simulink library "xps_library"  (Simulink 8.0)
settings: Solver=ode45  SolverMode=SingleTasking  StartTime=0.0  StopTime=10.0  RelTol=1e-3
undefined symbols (not defined in the file): sys_clk, xps_library_software_register_user_data_in
libraries: xbsIndex_r4 x867, simulink x109, dspsigops x81, casper_library_flow_control x68, xps_library x18, casper_library_misc x11
(part 10 of 10)

== system xps_library/DACs/dac_mkid/Subsystem/parallel_to_serial_converter ==
  pin : Inport
  ld : Inport  Port=2
  shift : Inport  Port=3
  Logical : xbsIndex_r4/Logical  logical_function=OR  inputs=2  en=off  latency=0  precision=Full  arith_type=Unsigned  n_bits=16  bin_pt=0  align_bp=on  dbl_ovrd=off  block_type=logical
  filler : xbsIndex_r4/Constant  const=0  gui_display_data_type=Fixed-point  arith_type=Unsigned  n_bits=sout_width  bin_pt=0  preci_type=Single  exp_width=8  frac_width=24  explicit_period=on  period=1  equ=P=C  opselect=C  inp2=PCIN>>17  opr=+  inp1=P  carry=CIN  dbl_ovrd=off  block_type=constant
  shifter_unit1 : casper_library_flow_control/shifter_unit  data_width=1  pin_offset=0
  shifter_unit10 : casper_library_flow_control/shifter_unit  data_width=1  pin_offset=9
  shifter_unit11 : casper_library_flow_control/shifter_unit  data_width=1  pin_offset=10
  shifter_unit12 : casper_library_flow_control/shifter_unit  data_width=1  pin_offset=11
  shifter_unit13 : casper_library_flow_control/shifter_unit  data_width=1  pin_offset=12
  shifter_unit14 : casper_library_flow_control/shifter_unit  data_width=1  pin_offset=13
  shifter_unit15 : casper_library_flow_control/shifter_unit  data_width=1  pin_offset=14
  shifter_unit16 : casper_library_flow_control/shifter_unit  data_width=1  pin_offset=15
  shifter_unit17 : casper_library_flow_control/shifter_unit  data_width=1  pin_offset=16
  shifter_unit2 : casper_library_flow_control/shifter_unit  data_width=1  pin_offset=1
  shifter_unit3 : casper_library_flow_control/shifter_unit  data_width=1  pin_offset=2
  shifter_unit4 : casper_library_flow_control/shifter_unit  data_width=1  pin_offset=3
  shifter_unit5 : casper_library_flow_control/shifter_unit  data_width=1  pin_offset=4
  shifter_unit6 : casper_library_flow_control/shifter_unit  data_width=1  pin_offset=5
  shifter_unit7 : casper_library_flow_control/shifter_unit  data_width=1  pin_offset=6
  shifter_unit8 : casper_library_flow_control/shifter_unit  data_width=1  pin_offset=7
  shifter_unit9 : casper_library_flow_control/shifter_unit  data_width=1  pin_offset=8
  sout : Outport
  wires:
  ld/1 -> Logical/1, shifter_unit1/1, shifter_unit2/1, shifter_unit3/1, shifter_unit4/1, shifter_unit5/1, shifter_unit6/1, shifter_unit7/1, shifter_unit8/1, shifter_unit9/1, shifter_unit10/1, shifter_unit11/1, shifter_unit12/1, shifter_unit13/1, shifter_unit14/1, shifter_unit15/1, shifter_unit16/1, shifter_unit17/1
  shift/1 -> Logical/2
  filler/1 -> shifter_unit1/2
  pin/1 -> shifter_unit1/3, shifter_unit2/3, shifter_unit3/3, shifter_unit4/3, shifter_unit5/3, shifter_unit6/3, shifter_unit7/3, shifter_unit8/3, shifter_unit9/3, shifter_unit10/3, shifter_unit11/3, shifter_unit12/3, shifter_unit13/3, shifter_unit14/3, shifter_unit15/3, shifter_unit16/3, shifter_unit17/3
  Logical/1 -> shifter_unit1/4, shifter_unit2/4, shifter_unit3/4, shifter_unit4/4, shifter_unit5/4, shifter_unit6/4, shifter_unit7/4, shifter_unit8/4, shifter_unit9/4, shifter_unit10/4, shifter_unit11/4, shifter_unit12/4, shifter_unit13/4, shifter_unit14/4, shifter_unit15/4, shifter_unit16/4, shifter_unit17/4
  shifter_unit1/1 -> shifter_unit2/2
  shifter_unit2/1 -> shifter_unit3/2
  shifter_unit3/1 -> shifter_unit4/2
  shifter_unit4/1 -> shifter_unit5/2
  shifter_unit5/1 -> shifter_unit6/2
  shifter_unit6/1 -> shifter_unit7/2
  shifter_unit7/1 -> shifter_unit8/2
  shifter_unit8/1 -> shifter_unit9/2
  shifter_unit9/1 -> shifter_unit10/2
  shifter_unit10/1 -> shifter_unit11/2
  shifter_unit11/1 -> shifter_unit12/2
  shifter_unit12/1 -> shifter_unit13/2
  shifter_unit13/1 -> shifter_unit14/2
  shifter_unit14/1 -> shifter_unit15/2
  shifter_unit15/1 -> shifter_unit16/2
  shifter_unit16/1 -> shifter_unit17/2
  shifter_unit17/1 -> sout/1

== system xps_library/DACs/dac_mkid/Subsystem/parallel_to_serial_converter1 ==
  pin : Inport
  ld : Inport  Port=2
  shift : Inport  Port=3
  Logical : xbsIndex_r4/Logical  logical_function=OR  inputs=2  en=off  latency=0  precision=Full  arith_type=Unsigned  n_bits=16  bin_pt=0  align_bp=on  dbl_ovrd=off  block_type=logical
  filler : xbsIndex_r4/Constant  const=0  gui_display_data_type=Fixed-point  arith_type=Unsigned  n_bits=sout_width  bin_pt=0  preci_type=Single  exp_width=8  frac_width=24  explicit_period=on  period=1  equ=P=C  opselect=C  inp2=PCIN>>17  opr=+  inp1=P  carry=CIN  dbl_ovrd=off  block_type=constant
  shifter_unit1 : casper_library_flow_control/shifter_unit  data_width=1  pin_offset=0
  shifter_unit10 : casper_library_flow_control/shifter_unit  data_width=1  pin_offset=9
  shifter_unit11 : casper_library_flow_control/shifter_unit  data_width=1  pin_offset=10
  shifter_unit12 : casper_library_flow_control/shifter_unit  data_width=1  pin_offset=11
  shifter_unit13 : casper_library_flow_control/shifter_unit  data_width=1  pin_offset=12
  shifter_unit14 : casper_library_flow_control/shifter_unit  data_width=1  pin_offset=13
  shifter_unit15 : casper_library_flow_control/shifter_unit  data_width=1  pin_offset=14
  shifter_unit16 : casper_library_flow_control/shifter_unit  data_width=1  pin_offset=15
  shifter_unit17 : casper_library_flow_control/shifter_unit  data_width=1  pin_offset=16
  shifter_unit2 : casper_library_flow_control/shifter_unit  data_width=1  pin_offset=1
  shifter_unit3 : casper_library_flow_control/shifter_unit  data_width=1  pin_offset=2
  shifter_unit4 : casper_library_flow_control/shifter_unit  data_width=1  pin_offset=3
  shifter_unit5 : casper_library_flow_control/shifter_unit  data_width=1  pin_offset=4
  shifter_unit6 : casper_library_flow_control/shifter_unit  data_width=1  pin_offset=5
  shifter_unit7 : casper_library_flow_control/shifter_unit  data_width=1  pin_offset=6
  shifter_unit8 : casper_library_flow_control/shifter_unit  data_width=1  pin_offset=7
  shifter_unit9 : casper_library_flow_control/shifter_unit  data_width=1  pin_offset=8
  sout : Outport
  wires:
  ld/1 -> Logical/1, shifter_unit1/1, shifter_unit2/1, shifter_unit3/1, shifter_unit4/1, shifter_unit5/1, shifter_unit6/1, shifter_unit7/1, shifter_unit8/1, shifter_unit9/1, shifter_unit10/1, shifter_unit11/1, shifter_unit12/1, shifter_unit13/1, shifter_unit14/1, shifter_unit15/1, shifter_unit16/1, shifter_unit17/1
  shift/1 -> Logical/2
  filler/1 -> shifter_unit1/2
  pin/1 -> shifter_unit1/3, shifter_unit2/3, shifter_unit3/3, shifter_unit4/3, shifter_unit5/3, shifter_unit6/3, shifter_unit7/3, shifter_unit8/3, shifter_unit9/3, shifter_unit10/3, shifter_unit11/3, shifter_unit12/3, shifter_unit13/3, shifter_unit14/3, shifter_unit15/3, shifter_unit16/3, shifter_unit17/3
  Logical/1 -> shifter_unit1/4, shifter_unit2/4, shifter_unit3/4, shifter_unit4/4, shifter_unit5/4, shifter_unit6/4, shifter_unit7/4, shifter_unit8/4, shifter_unit9/4, shifter_unit10/4, shifter_unit11/4, shifter_unit12/4, shifter_unit13/4, shifter_unit14/4, shifter_unit15/4, shifter_unit16/4, shifter_unit17/4
  shifter_unit1/1 -> shifter_unit2/2
  shifter_unit2/1 -> shifter_unit3/2
  shifter_unit3/1 -> shifter_unit4/2
  shifter_unit4/1 -> shifter_unit5/2
  shifter_unit5/1 -> shifter_unit6/2
  shifter_unit6/1 -> shifter_unit7/2
  shifter_unit7/1 -> shifter_unit8/2
  shifter_unit8/1 -> shifter_unit9/2
  shifter_unit9/1 -> shifter_unit10/2
  shifter_unit10/1 -> shifter_unit11/2
  shifter_unit11/1 -> shifter_unit12/2
  shifter_unit12/1 -> shifter_unit13/2
  shifter_unit13/1 -> shifter_unit14/2
  shifter_unit14/1 -> shifter_unit15/2
  shifter_unit15/1 -> shifter_unit16/2
  shifter_unit16/1 -> shifter_unit17/2
  shifter_unit17/1 -> sout/1

== system xps_library/DACs/dac_mkid/Subsystem/posedge1 ==
  In : Inport
  Delay : xbsIndex_r4/Delay  rst=off  infoeditControl=Selection of Reset will increase slice count due to use of real FFs and instead of SRLs  en=off  latency=1  dbl_ovrd=off  reg_retiming=off  block_type=delay
      settings: xl_area=[0, 0, 0, 0, 0, 0, 0]  block_version=9.1.01
  Inverter : xbsIndex_r4/Inverter  en=off  latency=0  dbl_ovrd=off  block_type=inv
      settings: xl_area=[0, 0, 0, 0, 0, 0, 0]  block_version=9.1.01
  Logical : xbsIndex_r4/Logical  logical_function=AND  inputs=2  en=off  latency=0  precision=Full  arith_type=Unsigned  n_bits=8  bin_pt=2  align_bp=on  dbl_ovrd=off  block_type=logical
      settings: xl_area=[0, 0, 0, 0, 0, 0, 0]  block_version=9.1.01
  Out : Outport
  wires:
  Delay/1 -> Inverter/1
  Inverter/1 -> Logical/1
  In/1 -> Delay/1, Logical/2
  Logical/1 -> Out/1

== system xps_library/DACs/dac_mkid/Subsystem/posedge2 ==
  In : Inport
  Delay : xbsIndex_r4/Delay  rst=off  infoeditControl=Selection of Reset will increase slice count due to use of real FFs and instead of SRLs  en=off  latency=1  dbl_ovrd=off  reg_retiming=off  block_type=delay
      settings: xl_area=[0, 0, 0, 0, 0, 0, 0]  block_version=9.1.01
  Inverter : xbsIndex_r4/Inverter  en=off  latency=0  dbl_ovrd=off  block_type=inv
      settings: xl_area=[0, 0, 0, 0, 0, 0, 0]  block_version=9.1.01
  Logical : xbsIndex_r4/Logical  logical_function=AND  inputs=2  en=off  latency=0  precision=Full  arith_type=Unsigned  n_bits=8  bin_pt=2  align_bp=on  dbl_ovrd=off  block_type=logical
      settings: xl_area=[0, 0, 0, 0, 0, 0, 0]  block_version=9.1.01
  Out : Outport
  wires:
  Delay/1 -> Inverter/1
  Inverter/1 -> Logical/1
  In/1 -> Delay/1, Logical/2
  Logical/1 -> Out/1

== system xps_library/DACs/dac_mkid/Subsystem/posedge3 ==
  In : Inport
  Delay : xbsIndex_r4/Delay  rst=off  infoeditControl=Selection of Reset will increase slice count due to use of real FFs and instead of SRLs  en=off  latency=1  dbl_ovrd=off  reg_retiming=off  block_type=delay
      settings: xl_area=[0, 0, 0, 0, 0, 0, 0]  block_version=9.1.01
  Inverter : xbsIndex_r4/Inverter  en=off  latency=0  dbl_ovrd=off  block_type=inv
      settings: xl_area=[0, 0, 0, 0, 0, 0, 0]  block_version=9.1.01
  Logical : xbsIndex_r4/Logical  logical_function=AND  inputs=2  en=off  latency=0  precision=Full  arith_type=Unsigned  n_bits=8  bin_pt=2  align_bp=on  dbl_ovrd=off  block_type=logical
      settings: xl_area=[0, 0, 0, 0, 0, 0, 0]  block_version=9.1.01
  Out : Outport
  wires:
  Delay/1 -> Inverter/1
  Inverter/1 -> Logical/1
  In/1 -> Delay/1, Logical/2
  Logical/1 -> Out/1

== system xps_library/DACs/dac_mkid_4x/Subsystem/parallel_to_serial_converter ==
  pin : Inport
  ld : Inport  Port=2
  shift : Inport  Port=3
  Logical : xbsIndex_r4/Logical  logical_function=OR  inputs=2  en=off  latency=0  precision=Full  arith_type=Unsigned  n_bits=16  bin_pt=0  align_bp=on  dbl_ovrd=off  block_type=logical
  filler : xbsIndex_r4/Constant  const=0  gui_display_data_type=Fixed-point  arith_type=Unsigned  n_bits=sout_width  bin_pt=0  preci_type=Single  exp_width=8  frac_width=24  explicit_period=on  period=1  equ=P=C  opselect=C  inp2=PCIN>>17  opr=+  inp1=P  carry=CIN  dbl_ovrd=off  block_type=constant
  shifter_unit1 : casper_library_flow_control/shifter_unit  data_width=1  pin_offset=0
  shifter_unit10 : casper_library_flow_control/shifter_unit  data_width=1  pin_offset=9
  shifter_unit11 : casper_library_flow_control/shifter_unit  data_width=1  pin_offset=10
  shifter_unit12 : casper_library_flow_control/shifter_unit  data_width=1  pin_offset=11
  shifter_unit13 : casper_library_flow_control/shifter_unit  data_width=1  pin_offset=12
  shifter_unit14 : casper_library_flow_control/shifter_unit  data_width=1  pin_offset=13
  shifter_unit15 : casper_library_flow_control/shifter_unit  data_width=1  pin_offset=14
  shifter_unit16 : casper_library_flow_control/shifter_unit  data_width=1  pin_offset=15
  shifter_unit17 : casper_library_flow_control/shifter_unit  data_width=1  pin_offset=16
  shifter_unit2 : casper_library_flow_control/shifter_unit  data_width=1  pin_offset=1
  shifter_unit3 : casper_library_flow_control/shifter_unit  data_width=1  pin_offset=2
  shifter_unit4 : casper_library_flow_control/shifter_unit  data_width=1  pin_offset=3
  shifter_unit5 : casper_library_flow_control/shifter_unit  data_width=1  pin_offset=4
  shifter_unit6 : casper_library_flow_control/shifter_unit  data_width=1  pin_offset=5
  shifter_unit7 : casper_library_flow_control/shifter_unit  data_width=1  pin_offset=6
  shifter_unit8 : casper_library_flow_control/shifter_unit  data_width=1  pin_offset=7
  shifter_unit9 : casper_library_flow_control/shifter_unit  data_width=1  pin_offset=8
  sout : Outport
  wires:
  shifter_unit17/1 -> sout/1
  shifter_unit16/1 -> shifter_unit17/2
  shifter_unit15/1 -> shifter_unit16/2
  shifter_unit14/1 -> shifter_unit15/2
  shifter_unit13/1 -> shifter_unit14/2
  shifter_unit12/1 -> shifter_unit13/2
  shifter_unit11/1 -> shifter_unit12/2
  shifter_unit10/1 -> shifter_unit11/2
  shifter_unit9/1 -> shifter_unit10/2
  shifter_unit8/1 -> shifter_unit9/2
  shifter_unit7/1 -> shifter_unit8/2
  shifter_unit6/1 -> shifter_unit7/2
  shifter_unit5/1 -> shifter_unit6/2
  shifter_unit4/1 -> shifter_unit5/2
  shifter_unit3/1 -> shifter_unit4/2
  shifter_unit2/1 -> shifter_unit3/2
  shifter_unit1/1 -> shifter_unit2/2
  Logical/1 -> shifter_unit17/4, shifter_unit16/4, shifter_unit15/4, shifter_unit14/4, shifter_unit13/4, shifter_unit12/4, shifter_unit11/4, shifter_unit10/4, shifter_unit9/4, shifter_unit8/4, shifter_unit7/4, shifter_unit6/4, shifter_unit5/4, shifter_unit4/4, shifter_unit3/4, shifter_unit2/4, shifter_unit1/4
  pin/1 -> shifter_unit17/3, shifter_unit16/3, shifter_unit15/3, shifter_unit14/3, shifter_unit13/3, shifter_unit12/3, shifter_unit11/3, shifter_unit10/3, shifter_unit9/3, shifter_unit8/3, shifter_unit7/3, shifter_unit6/3, shifter_unit5/3, shifter_unit4/3, shifter_unit3/3, shifter_unit2/3, shifter_unit1/3
  filler/1 -> shifter_unit1/2
  shift/1 -> Logical/2
  ld/1 -> shifter_unit17/1, shifter_unit16/1, shifter_unit15/1, shifter_unit14/1, shifter_unit13/1, shifter_unit12/1, shifter_unit11/1, shifter_unit10/1, shifter_unit9/1, shifter_unit8/1, shifter_unit7/1, shifter_unit6/1, shifter_unit5/1, shifter_unit4/1, shifter_unit3/1, shifter_unit2/1, shifter_unit1/1, Logical/1

== system xps_library/DACs/dac_mkid_4x/Subsystem/parallel_to_serial_converter1 ==
  pin : Inport
  ld : Inport  Port=2
  shift : Inport  Port=3
  Logical : xbsIndex_r4/Logical  logical_function=OR  inputs=2  en=off  latency=0  precision=Full  arith_type=Unsigned  n_bits=16  bin_pt=0  align_bp=on  dbl_ovrd=off  block_type=logical
  filler : xbsIndex_r4/Constant  const=0  gui_display_data_type=Fixed-point  arith_type=Unsigned  n_bits=sout_width  bin_pt=0  preci_type=Single  exp_width=8  frac_width=24  explicit_period=on  period=1  equ=P=C  opselect=C  inp2=PCIN>>17  opr=+  inp1=P  carry=CIN  dbl_ovrd=off  block_type=constant
  shifter_unit1 : casper_library_flow_control/shifter_unit  data_width=1  pin_offset=0
  shifter_unit10 : casper_library_flow_control/shifter_unit  data_width=1  pin_offset=9
  shifter_unit11 : casper_library_flow_control/shifter_unit  data_width=1  pin_offset=10
  shifter_unit12 : casper_library_flow_control/shifter_unit  data_width=1  pin_offset=11
  shifter_unit13 : casper_library_flow_control/shifter_unit  data_width=1  pin_offset=12
  shifter_unit14 : casper_library_flow_control/shifter_unit  data_width=1  pin_offset=13
  shifter_unit15 : casper_library_flow_control/shifter_unit  data_width=1  pin_offset=14
  shifter_unit16 : casper_library_flow_control/shifter_unit  data_width=1  pin_offset=15
  shifter_unit17 : casper_library_flow_control/shifter_unit  data_width=1  pin_offset=16
  shifter_unit2 : casper_library_flow_control/shifter_unit  data_width=1  pin_offset=1
  shifter_unit3 : casper_library_flow_control/shifter_unit  data_width=1  pin_offset=2
  shifter_unit4 : casper_library_flow_control/shifter_unit  data_width=1  pin_offset=3
  shifter_unit5 : casper_library_flow_control/shifter_unit  data_width=1  pin_offset=4
  shifter_unit6 : casper_library_flow_control/shifter_unit  data_width=1  pin_offset=5
  shifter_unit7 : casper_library_flow_control/shifter_unit  data_width=1  pin_offset=6
  shifter_unit8 : casper_library_flow_control/shifter_unit  data_width=1  pin_offset=7
  shifter_unit9 : casper_library_flow_control/shifter_unit  data_width=1  pin_offset=8
  sout : Outport
  wires:
  shifter_unit17/1 -> sout/1
  shifter_unit16/1 -> shifter_unit17/2
  shifter_unit15/1 -> shifter_unit16/2
  shifter_unit14/1 -> shifter_unit15/2
  shifter_unit13/1 -> shifter_unit14/2
  shifter_unit12/1 -> shifter_unit13/2
  shifter_unit11/1 -> shifter_unit12/2
  shifter_unit10/1 -> shifter_unit11/2
  shifter_unit9/1 -> shifter_unit10/2
  shifter_unit8/1 -> shifter_unit9/2
  shifter_unit7/1 -> shifter_unit8/2
  shifter_unit6/1 -> shifter_unit7/2
  shifter_unit5/1 -> shifter_unit6/2
  shifter_unit4/1 -> shifter_unit5/2
  shifter_unit3/1 -> shifter_unit4/2
  shifter_unit2/1 -> shifter_unit3/2
  shifter_unit1/1 -> shifter_unit2/2
  Logical/1 -> shifter_unit17/4, shifter_unit16/4, shifter_unit15/4, shifter_unit14/4, shifter_unit13/4, shifter_unit12/4, shifter_unit11/4, shifter_unit10/4, shifter_unit9/4, shifter_unit8/4, shifter_unit7/4, shifter_unit6/4, shifter_unit5/4, shifter_unit4/4, shifter_unit3/4, shifter_unit2/4, shifter_unit1/4
  pin/1 -> shifter_unit17/3, shifter_unit16/3, shifter_unit15/3, shifter_unit14/3, shifter_unit13/3, shifter_unit12/3, shifter_unit11/3, shifter_unit10/3, shifter_unit9/3, shifter_unit8/3, shifter_unit7/3, shifter_unit6/3, shifter_unit5/3, shifter_unit4/3, shifter_unit3/3, shifter_unit2/3, shifter_unit1/3
  filler/1 -> shifter_unit1/2
  shift/1 -> Logical/2
  ld/1 -> shifter_unit17/1, shifter_unit16/1, shifter_unit15/1, shifter_unit14/1, shifter_unit13/1, shifter_unit12/1, shifter_unit11/1, shifter_unit10/1, shifter_unit9/1, shifter_unit8/1, shifter_unit7/1, shifter_unit6/1, shifter_unit5/1, shifter_unit4/1, shifter_unit3/1, shifter_unit2/1, shifter_unit1/1, Logical/1

== system xps_library/DACs/dac_mkid_4x/Subsystem/posedge1 ==
  In : Inport
  Delay : xbsIndex_r4/Delay  rst=off  infoeditControl=Selection of Reset will increase slice count due to use of real FFs and instead of SRLs  en=off  latency=1  dbl_ovrd=off  reg_retiming=off  block_type=delay
      settings: xl_area=[0, 0, 0, 0, 0, 0, 0]  block_version=9.1.01
  Inverter : xbsIndex_r4/Inverter  en=off  latency=0  dbl_ovrd=off  block_type=inv
      settings: xl_area=[0, 0, 0, 0, 0, 0, 0]  block_version=9.1.01
  Logical : xbsIndex_r4/Logical  logical_function=AND  inputs=2  en=off  latency=0  precision=Full  arith_type=Unsigned  n_bits=8  bin_pt=2  align_bp=on  dbl_ovrd=off  block_type=logical
      settings: xl_area=[0, 0, 0, 0, 0, 0, 0]  block_version=9.1.01
  Out : Outport
  wires:
  Logical/1 -> Out/1
  In/1 -> Logical/2, Delay/1
  Inverter/1 -> Logical/1
  Delay/1 -> Inverter/1

== system xps_library/DACs/dac_mkid_4x/Subsystem/posedge2 ==
  In : Inport
  Delay : xbsIndex_r4/Delay  rst=off  infoeditControl=Selection of Reset will increase slice count due to use of real FFs and instead of SRLs  en=off  latency=1  dbl_ovrd=off  reg_retiming=off  block_type=delay
      settings: xl_area=[0, 0, 0, 0, 0, 0, 0]  block_version=9.1.01
  Inverter : xbsIndex_r4/Inverter  en=off  latency=0  dbl_ovrd=off  block_type=inv
      settings: xl_area=[0, 0, 0, 0, 0, 0, 0]  block_version=9.1.01
  Logical : xbsIndex_r4/Logical  logical_function=AND  inputs=2  en=off  latency=0  precision=Full  arith_type=Unsigned  n_bits=8  bin_pt=2  align_bp=on  dbl_ovrd=off  block_type=logical
      settings: xl_area=[0, 0, 0, 0, 0, 0, 0]  block_version=9.1.01
  Out : Outport
  wires:
  Logical/1 -> Out/1
  In/1 -> Logical/2, Delay/1
  Inverter/1 -> Logical/1
  Delay/1 -> Inverter/1

== system xps_library/DACs/dac_mkid_4x/Subsystem/posedge3 ==
  In : Inport
  Delay : xbsIndex_r4/Delay  rst=off  infoeditControl=Selection of Reset will increase slice count due to use of real FFs and instead of SRLs  en=off  latency=1  dbl_ovrd=off  reg_retiming=off  block_type=delay
      settings: xl_area=[0, 0, 0, 0, 0, 0, 0]  block_version=9.1.01
  Inverter : xbsIndex_r4/Inverter  en=off  latency=0  dbl_ovrd=off  block_type=inv
      settings: xl_area=[0, 0, 0, 0, 0, 0, 0]  block_version=9.1.01
  Logical : xbsIndex_r4/Logical  logical_function=AND  inputs=2  en=off  latency=0  precision=Full  arith_type=Unsigned  n_bits=8  bin_pt=2  align_bp=on  dbl_ovrd=off  block_type=logical
      settings: xl_area=[0, 0, 0, 0, 0, 0, 0]  block_version=9.1.01
  Out : Outport
  wires:
  Logical/1 -> Out/1
  In/1 -> Logical/2, Delay/1
  Inverter/1 -> Logical/1
  Delay/1 -> Inverter/1
